simulink model "Z2"  (R2023b)
settings: Solver=VariableStepAuto  StartTime=0.0  StopTime=10  RelTol=1e-3
settings Model: Creator=Liu  LastModifiedBy=Liu

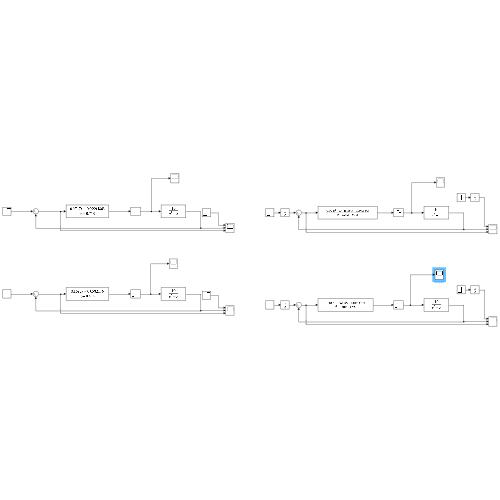
[thumbnail: Simulink's stored preview of the top-level diagram]
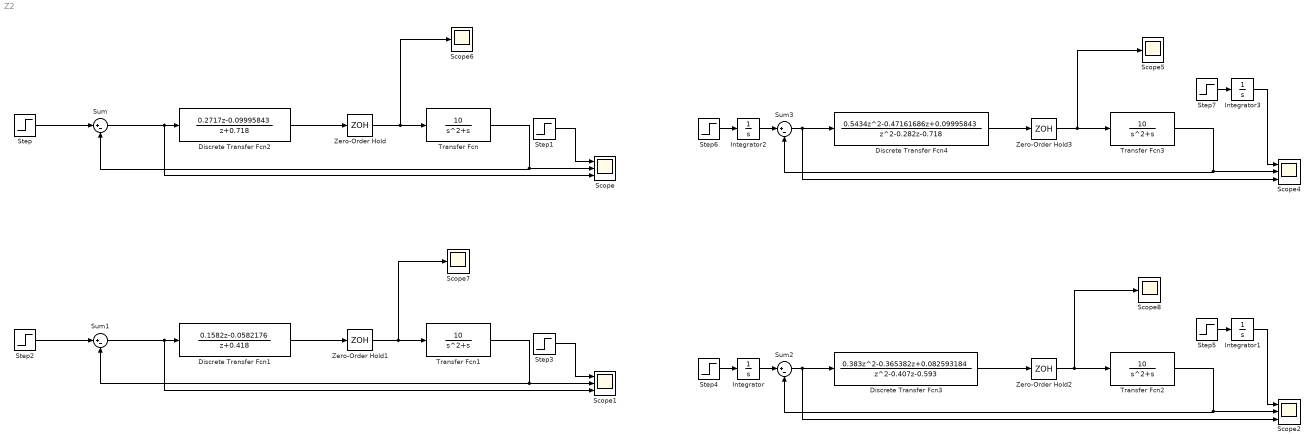
== system Z2 ==
  Discrete Transfer Fcn1 : DiscreteTransferFcn  Numerator=[0.1582 -0.0582176]  Denominator=[1 0.418]
  Discrete Transfer Fcn2 : DiscreteTransferFcn  Numerator=[0.2717 -0.09995843]  Denominator=[1 0.718]
  Discrete Transfer Fcn3 : DiscreteTransferFcn  Numerator=[0.383 -0.365382 0.082593184]  Denominator=[1 -0.407 -0.593]
  Discrete Transfer Fcn4 : DiscreteTransferFcn  Numerator=[0.5434 -0.47161686 0.09995843]  Denominator=[1 -0.282 -0.718]
  Integrator{,1..3} (4 alike) : Integrator
  Scope{,1..2,4} (4 alike) : Scope  NumInputPorts=3
  Scope{5..8} (4 alike) : Scope
  Step{,1..7} (8 alike) : Step  Time=0  SampleTime=0
  Sum{,1..3} (4 alike) : Sum  Inputs=|+-
  Transfer Fcn{,1..3} (4 alike) : TransferFcn  Numerator=[0 10]  Denominator=[1 1 0]
  Zero-Order Hold{,1..3} (4 alike) : ZeroOrderHold
  wires:
  Step/1 -> Sum/1
  Zero-Order Hold/1 -> Scope6/1, Transfer Fcn/1
  Transfer Fcn/1 -> Sum/2, Scope/2
  Discrete Transfer Fcn2/1 -> Zero-Order Hold/1
  Step1/1 -> Scope/1
  Sum/1 -> Discrete Transfer Fcn2/1, Scope/3
  Sum1/1 -> Discrete Transfer Fcn1/1, Scope1/3
  Discrete Transfer Fcn1/1 -> Zero-Order Hold1/1
  Transfer Fcn1/1 -> Sum1/2, Scope1/2
  Step3/1 -> Scope1/1
  Step2/1 -> Sum1/1
  Sum2/1 -> Discrete Transfer Fcn3/1, Scope2/3
  Discrete Transfer Fcn3/1 -> Zero-Order Hold2/1
  Transfer Fcn2/1 -> Sum2/2, Scope2/2
  Step4/1 -> Integrator/1
  Integrator/1 -> Sum2/1
  Step5/1 -> Integrator1/1
  Integrator1/1 -> Scope2/1
  Integrator2/1 -> Sum3/1
  Step6/1 -> Integrator2/1
  Discrete Transfer Fcn4/1 -> Zero-Order Hold3/1
  Transfer Fcn3/1 -> Sum3/2, Scope4/2
  Integrator3/1 -> Scope4/1
  Sum3/1 -> Discrete Transfer Fcn4/1, Scope4/3
  Step7/1 -> Integrator3/1
  Zero-Order Hold1/1 -> Scope7/1, Transfer Fcn1/1
  Zero-Order Hold3/1 -> Scope5/1, Transfer Fcn3/1
  Zero-Order Hold2/1 -> Scope8/1, Transfer Fcn2/1
